simulink model "breakdown_FF"  (R2022b)
settings: Solver=VariableStepAuto  StartTime=0.0  StopTime=10.0  RelTol=1e-3
PreLoadFcn:
  | TOP;
undefined symbols (not defined in the file): ff_p, ff_z, p, r
libraries: dsparch4 x9, dspsrcs4 x4, dspspect3 x3, simulink_extras x3, dspmathops x3, cstblocks x2
settings Model: SimulationMode=accelerator  Creator=kschutz  LastModifiedBy=kschutz

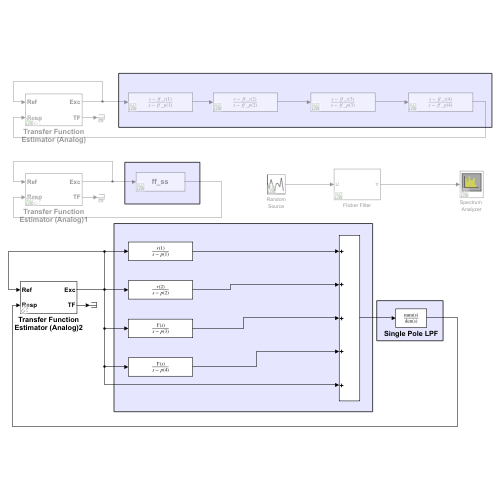
[thumbnail: Simulink's stored preview of the top-level diagram]
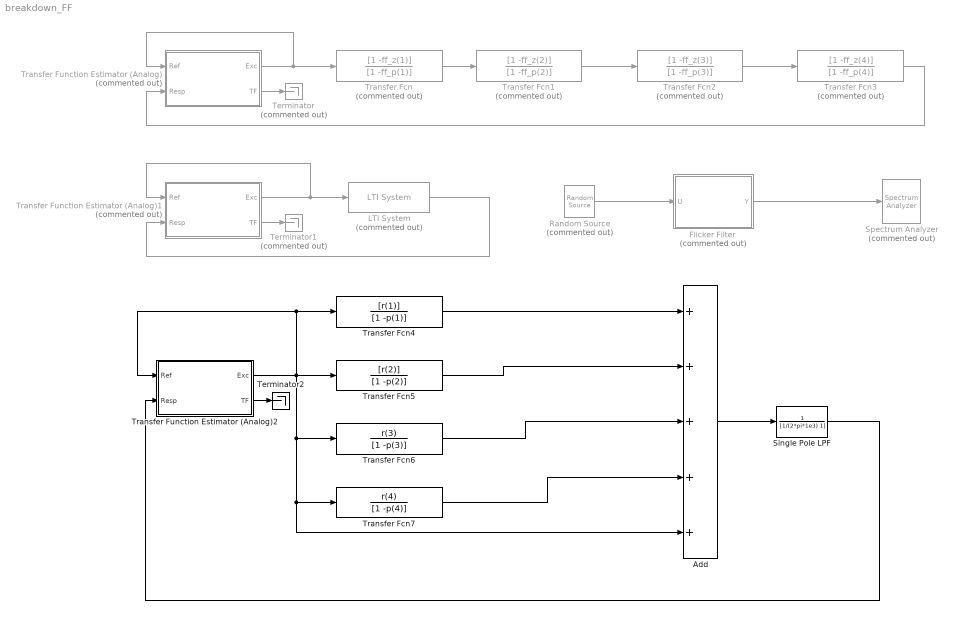
== system breakdown_FF ==
  Add : Sum  Inputs=+++++
  Flicker Filter : Subsystem  Commented=on
  LTI System : cstblocks/LTI System  Commented=on  sys=ff_ss  IC=[]
  Random Source : dspsrcs4/Random Source  Commented=on  SrcType=Uniform  NormMethod=Ziggurat  CltLength=12  MinVal=0  MaxVal=1  MeanVal=0  VarVal=1  RepMode=Not repeatable  rawSeed=1  IsInherit=off  SampMode=Discrete  SampTime=1e-5  SampFrame=1  DataType=Double  OutComplex=Real  OutputFrames=off
  Single Pole LPF : TransferFcn  Denominator=[1/(2*pi*1e3) 1]
  Spectrum Analyzer : SpectrumAnalyzer  Commented=on
  Terminator : Terminator  Commented=on
  Terminator1 : Terminator  Commented=on
  Terminator2 : Terminator
  Transfer Fcn : TransferFcn  Commented=on  Numerator=[1 -ff_z(1)]  Denominator=[1 -ff_p(1)]
  Transfer Fcn1 : TransferFcn  Commented=on  Numerator=[1 -ff_z(2)]  Denominator=[1 -ff_p(2)]
  Transfer Fcn2 : TransferFcn  Commented=on  Numerator=[1 -ff_z(3)]  Denominator=[1 -ff_p(3)]
  Transfer Fcn3 : TransferFcn  Commented=on  Numerator=[1 -ff_z(4)]  Denominator=[1 -ff_p(4)]
  Transfer Fcn4 : TransferFcn  Numerator=[r(1)]  Denominator=[1 -p(1)]
  Transfer Fcn5 : TransferFcn  Numerator=[r(2)]  Denominator=[1 -p(2)]
  Transfer Fcn6 : TransferFcn  Numerator=r(3)  Denominator=[1 -p(3)]
  Transfer Fcn7 : TransferFcn  Numerator=r(4)  Denominator=[1 -p(4)]
  Transfer Function Estimator (Analog) : Subsystem  Commented=on  AncestorBlock=|  mask(Baseband Analog Transfer Function Estimator){BW=100e3, Nfft=100e3, Navg=1, HoldOff=0}
      | Kblocks/Transfer Function
      | Estimator (Analog)
      mask prompts: BW "Bandwidth"; Nfft "FFT size"; Navg "Number of Averages"; HoldOff "Hold Off (seconds)"
      mask init:
      | % Select subset of FFT bins that are not aliased
      | % for output and display purposes.
      | % Said subset is based on the oversampling factor.
      | % Here we use a 2.56x oversampling factor.
      | % For example, for a 1024 point FFT size, the relatively
      | % alias free FFT bins would be bins 1 to 401.
      | % floor(1024/2.56) + 1 = 401.
      | OSR = 2.56;
      | AliasFree = floor(Nfft/OSR) + 1;
      settings: LibrarySourceBlock=|
      | Kblocks/Transfer Function
      | Estimator (Analog)
  Transfer Function Estimator (Analog)1 : Subsystem  Commented=on  AncestorBlock=|  mask(Baseband Analog Transfer Function Estimator){BW=100e3, Nfft=100e3, Navg=1, HoldOff=0}
      | Kblocks/Transfer Function
      | Estimator (Analog)
      mask prompts: BW "Bandwidth"; Nfft "FFT size"; Navg "Number of Averages"; HoldOff "Hold Off (seconds)"
      mask init: same as breakdown_FF/Transfer Function Estimator (Analog)
      settings: LibrarySourceBlock=|
      | Kblocks/Transfer Function
      | Estimator (Analog)
  Transfer Function Estimator (Analog)2 : Subsystem  AncestorBlock=|  mask(Baseband Analog Transfer Function Estimator){BW=100e3, Nfft=100e3, Navg=1, HoldOff=0}
      | Kblocks/Transfer Function
      | Estimator (Analog)
      mask prompts: BW "Bandwidth"; Nfft "FFT size"; Navg "Number of Averages"; HoldOff "Hold Off (seconds)"
      mask init: same as breakdown_FF/Transfer Function Estimator (Analog)
      settings: LibrarySourceBlock=|
      | Kblocks/Transfer Function
      | Estimator (Analog)
  wires:
  Transfer Fcn/1 -> Transfer Fcn1/1
  Transfer Fcn1/1 -> Transfer Fcn2/1
  Transfer Fcn2/1 -> Transfer Fcn3/1
  Transfer Function Estimator (Analog)/1(Exc) -> Transfer Function Estimator (Analog)/1(Ref), Transfer Fcn/1
  Transfer Fcn3/1 -> Transfer Function Estimator (Analog)/2(Resp)
  Transfer Function Estimator (Analog)1/1(Exc) -> Transfer Function Estimator (Analog)1/1(Ref), LTI System/1
  LTI System/1 -> Transfer Function Estimator (Analog)1/2(Resp)
  Transfer Function Estimator (Analog)2/1(Exc) -> Transfer Fcn7/1, Add/5, Transfer Fcn6/1, Transfer Fcn5/1, Transfer Fcn4/1, Transfer Function Estimator (Analog)2/1(Ref)
  Transfer Fcn4/1 -> Add/1
  Transfer Fcn5/1 -> Add/2
  Transfer Fcn6/1 -> Add/3
  Transfer Fcn7/1 -> Add/4
  Add/1 -> Single Pole LPF/1
  Single Pole LPF/1 -> Transfer Function Estimator (Analog)2/2(Resp)
  Transfer Function Estimator (Analog)/2(TF) -> Terminator/1
  Transfer Function Estimator (Analog)1/2(TF) -> Terminator1/1
  Transfer Function Estimator (Analog)2/2(TF) -> Terminator2/1
  Random Source/1 -> Flicker Filter/1(U)
  Flicker Filter/1(Y) -> Spectrum Analyzer/1

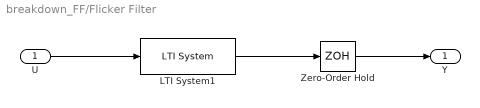
== system breakdown_FF/Flicker Filter ==
  U : Inport
  LTI System1 : cstblocks/LTI System  sys=ff_ss  IC=[]
  Zero-Order Hold : ZeroOrderHold  SampleTime=1e-5
  Y : Outport
  wires:
  Zero-Order Hold/1 -> Y/1
  LTI System1/1 -> Zero-Order Hold/1
  U/1 -> LTI System1/1

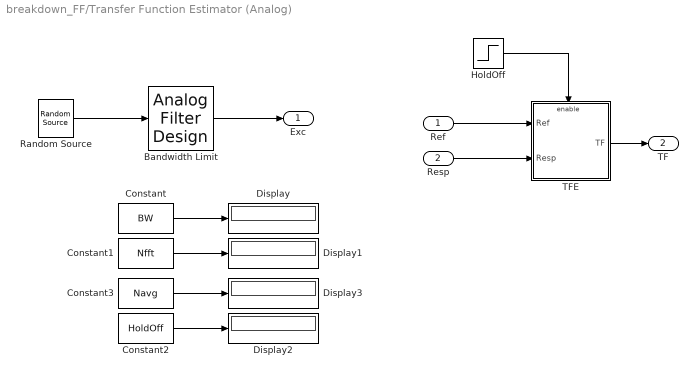
== system breakdown_FF/Transfer Function Estimator (Analog) ==
  Ref : Inport
  Resp : Inport  Port=2
  Bandwidth Limit : dsparch4/Analog Filter Design  method=Elliptic  filttype=Lowpass  N=8  Wlo=2*pi*BW  Whi=80  Rp=2  Rs=120
  Constant : Constant  Value=BW
  Constant1 : Constant  Value=Nfft
  Constant2 : Constant  Value=HoldOff
  Constant3 : Constant  Value=Navg
  Display{,1..3} (4 alike) : Display
  HoldOff : Step  Time=HoldOff  SampleTime=0
  Random Source : dspsrcs4/Random Source  SrcType=Uniform  NormMethod=Ziggurat  CltLength=12  MinVal=0  MaxVal=1  MeanVal=0  VarVal=1  RepMode=Specify seed  rawSeed=1  IsInherit=off  SampMode=Discrete  SampTime=1/(2.56*BW)  SampFrame=1  DataType=Double  OutComplex=Real  OutputFrames=off
  TFE : Subsystem
  Exc : Outport
  TF : Outport  Port=2
  wires:
  TFE/1(TF) -> TF/1
  Bandwidth Limit/1 -> Exc/1
  Random Source/1 -> Bandwidth Limit/1
  Constant1/1 -> Display1/1
  Constant2/1 -> Display2/1
  Constant/1 -> Display/1
  Ref/1 -> TFE/1(Ref)
  Resp/1 -> TFE/2(Resp)
  HoldOff/1 -> TFE/Enable
  Constant3/1 -> Display3/1

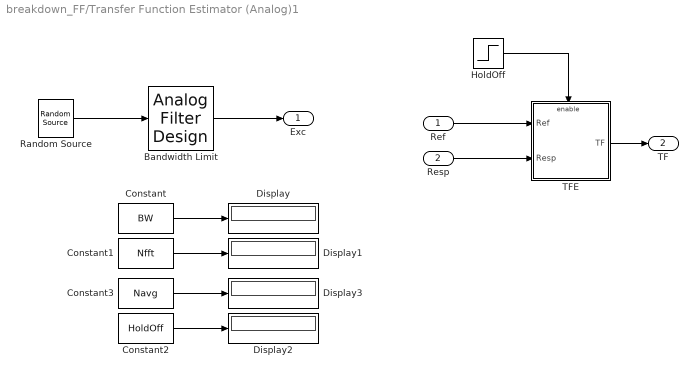
== system breakdown_FF/Transfer Function Estimator (Analog)1 ==
  Ref : Inport
  Resp : Inport  Port=2
  Bandwidth Limit : dsparch4/Analog Filter Design  method=Elliptic  filttype=Lowpass  N=8  Wlo=2*pi*BW  Whi=80  Rp=2  Rs=120
  Constant : Constant  Value=BW
  Constant1 : Constant  Value=Nfft
  Constant2 : Constant  Value=HoldOff
  Constant3 : Constant  Value=Navg
  Display{,1..3} (4 alike) : Display
  HoldOff : Step  Time=HoldOff  SampleTime=0
  Random Source : dspsrcs4/Random Source  SrcType=Uniform  NormMethod=Ziggurat  CltLength=12  MinVal=0  MaxVal=1  MeanVal=0  VarVal=1  RepMode=Specify seed  rawSeed=1  IsInherit=off  SampMode=Discrete  SampTime=1/(2.56*BW)  SampFrame=1  DataType=Double  OutComplex=Real  OutputFrames=off
  TFE : Subsystem
  Exc : Outport
  TF : Outport  Port=2
  wires:
  Constant3/1 -> Display3/1
  HoldOff/1 -> TFE/Enable
  Resp/1 -> TFE/2(Resp)
  Ref/1 -> TFE/1(Ref)
  Constant/1 -> Display/1
  Constant2/1 -> Display2/1
  Constant1/1 -> Display1/1
  Random Source/1 -> Bandwidth Limit/1
  Bandwidth Limit/1 -> Exc/1
  TFE/1(TF) -> TF/1

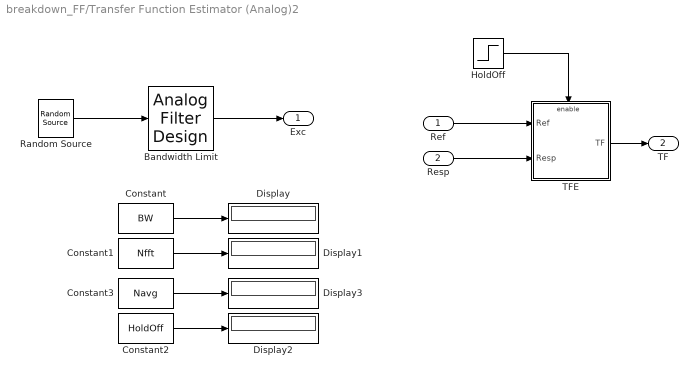
== system breakdown_FF/Transfer Function Estimator (Analog)2 ==
  Ref : Inport
  Resp : Inport  Port=2
  Bandwidth Limit : dsparch4/Analog Filter Design  method=Elliptic  filttype=Lowpass  N=8  Wlo=2*pi*BW  Whi=80  Rp=2  Rs=120
  Constant : Constant  Value=BW
  Constant1 : Constant  Value=Nfft
  Constant2 : Constant  Value=HoldOff
  Constant3 : Constant  Value=Navg
  Display{,1..3} (4 alike) : Display
  HoldOff : Step  Time=HoldOff  SampleTime=0
  Random Source : dspsrcs4/Random Source  SrcType=Uniform  NormMethod=Ziggurat  CltLength=12  MinVal=0  MaxVal=1  MeanVal=0  VarVal=1  RepMode=Specify seed  rawSeed=1  IsInherit=off  SampMode=Discrete  SampTime=1/(2.56*BW)  SampFrame=1  DataType=Double  OutComplex=Real  OutputFrames=off
  TFE : Subsystem
  Exc : Outport
  TF : Outport  Port=2
  wires:
  TFE/1(TF) -> TF/1
  Bandwidth Limit/1 -> Exc/1
  Random Source/1 -> Bandwidth Limit/1
  Constant1/1 -> Display1/1
  Constant2/1 -> Display2/1
  Constant/1 -> Display/1
  Ref/1 -> TFE/1(Ref)
  Resp/1 -> TFE/2(Resp)
  HoldOff/1 -> TFE/Enable
  Constant3/1 -> Display3/1

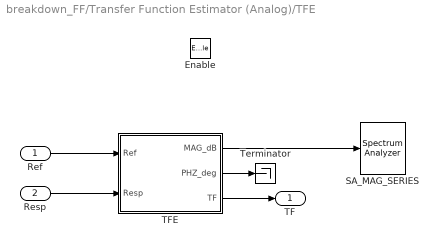
== system breakdown_FF/Transfer Function Estimator (Analog)/TFE ==
  Ref : Inport
  Resp : Inport  Port=2
  Enable : EnablePort
  SA_MAG_SERIES : SpectrumAnalyzer  IsFrequencyInputMode=1
  TFE : Subsystem
  Terminator : Terminator
  TF : Outport
  wires:
  TFE/3(TF) -> TF/1
  Resp/1 -> TFE/2(Resp)
  Ref/1 -> TFE/1(Ref)
  TFE/1(MAG_dB) -> SA_MAG_SERIES/1
  TFE/2(PHZ_deg) -> Terminator/1

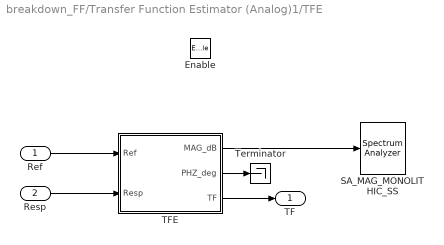
== system breakdown_FF/Transfer Function Estimator (Analog)1/TFE ==
  Ref : Inport
  Resp : Inport  Port=2
  Enable : EnablePort
  SA_MAG_MONOLITHIC_SS : SpectrumAnalyzer  IsFrequencyInputMode=1
  TFE : Subsystem
  Terminator : Terminator
  TF : Outport
  wires:
  TFE/1(MAG_dB) -> SA_MAG_MONOLITHIC_SS/1
  Ref/1 -> TFE/1(Ref)
  Resp/1 -> TFE/2(Resp)
  TFE/3(TF) -> TF/1
  TFE/2(PHZ_deg) -> Terminator/1

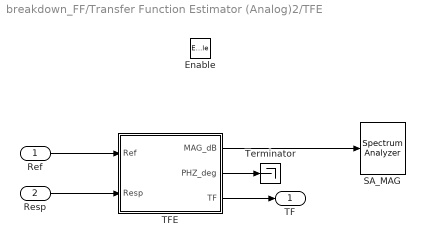
== system breakdown_FF/Transfer Function Estimator (Analog)2/TFE ==
  Ref : Inport
  Resp : Inport  Port=2
  Enable : EnablePort
  SA_MAG : SpectrumAnalyzer  IsFrequencyInputMode=1
  TFE : Subsystem
  Terminator : Terminator
  TF : Outport
  wires:
  TFE/3(TF) -> TF/1
  Resp/1 -> TFE/2(Resp)
  Ref/1 -> TFE/1(Ref)
  TFE/1(MAG_dB) -> SA_MAG/1
  TFE/2(PHZ_deg) -> Terminator/1

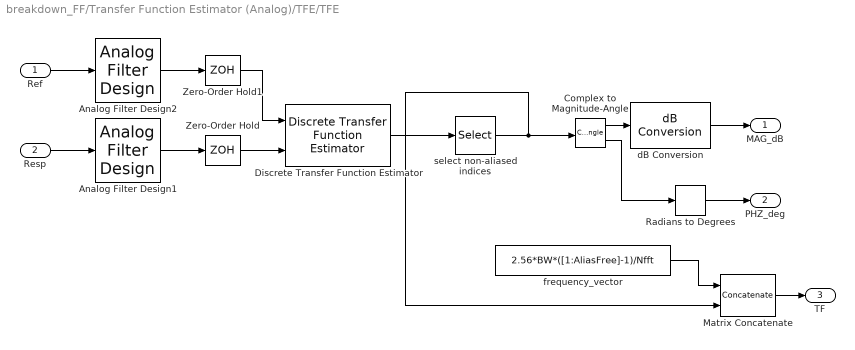
== system breakdown_FF/Transfer Function Estimator (Analog)/TFE/TFE ==
  Ref : Inport
  Resp : Inport  Port=2
  Analog Filter Design1 : dsparch4/Analog Filter Design  method=Elliptic  filttype=Lowpass  N=8  Wlo=2*pi*BW  Whi=80  Rp=2  Rs=100
  Analog Filter Design2 : dsparch4/Analog Filter Design  method=Elliptic  filttype=Lowpass  N=8  Wlo=2*pi*BW  Whi=80  Rp=2  Rs=100
  Complex to Magnitude-Angle : ComplexToMagnitudeAngle
  Discrete Transfer Function Estimator : dspspect3/Discrete Transfer Function Estimator  WindowMode=Specify on dialog  WindowLength=Nfft  Overlap=0  AveragingMethod=Running  ForgettingFactorPort=off  ForgettingFactor=0.9  SpectralAverages=Navg  FFTLengthSource=Property  FFTLength=Nfft  Window=Hann  SidelobeAttenuation=60  FrequencyRange=One-sided  OutputCoherence=off  SimulateUsing=Interpreted execution
  Matrix Concatenate : Concatenate  Mode=Multidimensional array  ConcatenateDimension=2
  Radians to Degrees : simulink_extras/Transformations/Radians to Degrees
  Zero-Order Hold : ZeroOrderHold  SampleTime=1/(OSR*BW)
  Zero-Order Hold1 : ZeroOrderHold  SampleTime=1/(OSR*BW)
  dB Conversion : dspmathops/dB Conversion  dBtype=dB  intype=Amplitude  R=1  fuzz=off
  frequency_vector : Constant  Value=2.56*BW*([1:AliasFree]-1)/Nfft
  select non-aliased indices : Selector  NumberOfDimensions=2  InputPortWidth=3  IndexOptions=Index vector (dialog),Select all  Indices=[1:AliasFree ],1  OutputSizes=1,1
  MAG_dB : Outport
  PHZ_deg : Outport  Port=2
  TF : Outport  Port=3
  wires:
  Matrix Concatenate/1 -> TF/1
  select non-aliased indices/1 -> Complex to Magnitude-Angle/1, Matrix Concatenate/2
  frequency_vector/1 -> Matrix Concatenate/1
  Discrete Transfer Function Estimator/1 -> select non-aliased indices/1
  Complex to Magnitude-Angle/2 -> Radians to Degrees/1
  Analog Filter Design1/1 -> Zero-Order Hold/1
  Analog Filter Design2/1 -> Zero-Order Hold1/1
  Radians to Degrees/1 -> PHZ_deg/1
  dB Conversion/1 -> MAG_dB/1
  Resp/1 -> Analog Filter Design1/1
  Zero-Order Hold1/1 -> Discrete Transfer Function Estimator/1
  Ref/1 -> Analog Filter Design2/1
  Complex to Magnitude-Angle/1 -> dB Conversion/1
  Zero-Order Hold/1 -> Discrete Transfer Function Estimator/2

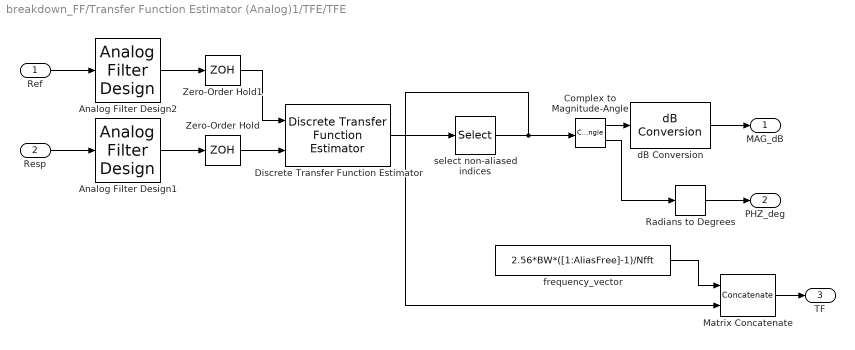
== system breakdown_FF/Transfer Function Estimator (Analog)1/TFE/TFE ==
  Ref : Inport
  Resp : Inport  Port=2
  Analog Filter Design1 : dsparch4/Analog Filter Design  method=Elliptic  filttype=Lowpass  N=8  Wlo=2*pi*BW  Whi=80  Rp=2  Rs=100
  Analog Filter Design2 : dsparch4/Analog Filter Design  method=Elliptic  filttype=Lowpass  N=8  Wlo=2*pi*BW  Whi=80  Rp=2  Rs=100
  Complex to Magnitude-Angle : ComplexToMagnitudeAngle
  Discrete Transfer Function Estimator : dspspect3/Discrete Transfer Function Estimator  WindowMode=Specify on dialog  WindowLength=Nfft  Overlap=0  AveragingMethod=Running  ForgettingFactorPort=off  ForgettingFactor=0.9  SpectralAverages=Navg  FFTLengthSource=Property  FFTLength=Nfft  Window=Hann  SidelobeAttenuation=60  FrequencyRange=One-sided  OutputCoherence=off  SimulateUsing=Interpreted execution
  Matrix Concatenate : Concatenate  Mode=Multidimensional array  ConcatenateDimension=2
  Radians to Degrees : simulink_extras/Transformations/Radians to Degrees
  Zero-Order Hold : ZeroOrderHold  SampleTime=1/(OSR*BW)
  Zero-Order Hold1 : ZeroOrderHold  SampleTime=1/(OSR*BW)
  dB Conversion : dspmathops/dB Conversion  dBtype=dB  intype=Amplitude  R=1  fuzz=off
  frequency_vector : Constant  Value=2.56*BW*([1:AliasFree]-1)/Nfft
  select non-aliased indices : Selector  NumberOfDimensions=2  InputPortWidth=3  IndexOptions=Index vector (dialog),Select all  Indices=[1:AliasFree ],1  OutputSizes=1,1
  MAG_dB : Outport
  PHZ_deg : Outport  Port=2
  TF : Outport  Port=3
  wires:
  Zero-Order Hold/1 -> Discrete Transfer Function Estimator/2
  Complex to Magnitude-Angle/1 -> dB Conversion/1
  Ref/1 -> Analog Filter Design2/1
  Zero-Order Hold1/1 -> Discrete Transfer Function Estimator/1
  Resp/1 -> Analog Filter Design1/1
  dB Conversion/1 -> MAG_dB/1
  Radians to Degrees/1 -> PHZ_deg/1
  Analog Filter Design2/1 -> Zero-Order Hold1/1
  Analog Filter Design1/1 -> Zero-Order Hold/1
  Complex to Magnitude-Angle/2 -> Radians to Degrees/1
  Discrete Transfer Function Estimator/1 -> select non-aliased indices/1
  frequency_vector/1 -> Matrix Concatenate/1
  select non-aliased indices/1 -> Matrix Concatenate/2, Complex to Magnitude-Angle/1
  Matrix Concatenate/1 -> TF/1

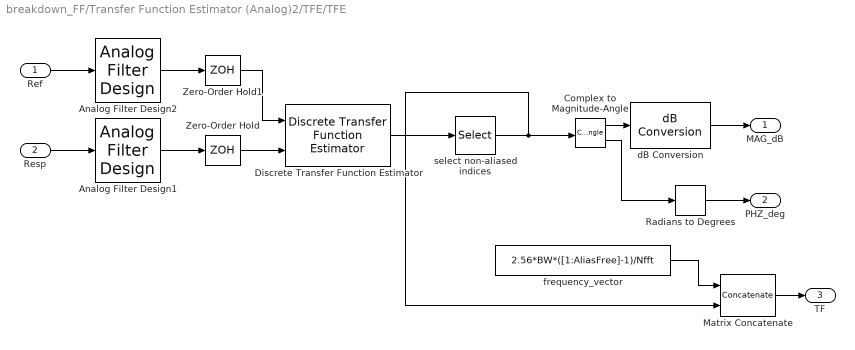
== system breakdown_FF/Transfer Function Estimator (Analog)2/TFE/TFE ==
  Ref : Inport
  Resp : Inport  Port=2
  Analog Filter Design1 : dsparch4/Analog Filter Design  method=Elliptic  filttype=Lowpass  N=8  Wlo=2*pi*BW  Whi=80  Rp=2  Rs=100
  Analog Filter Design2 : dsparch4/Analog Filter Design  method=Elliptic  filttype=Lowpass  N=8  Wlo=2*pi*BW  Whi=80  Rp=2  Rs=100
  Complex to Magnitude-Angle : ComplexToMagnitudeAngle
  Discrete Transfer Function Estimator : dspspect3/Discrete Transfer Function Estimator  WindowMode=Specify on dialog  WindowLength=Nfft  Overlap=0  AveragingMethod=Running  ForgettingFactorPort=off  ForgettingFactor=0.9  SpectralAverages=Navg  FFTLengthSource=Property  FFTLength=Nfft  Window=Hann  SidelobeAttenuation=60  FrequencyRange=One-sided  OutputCoherence=off  SimulateUsing=Interpreted execution
  Matrix Concatenate : Concatenate  Mode=Multidimensional array  ConcatenateDimension=2
  Radians to Degrees : simulink_extras/Transformations/Radians to Degrees
  Zero-Order Hold : ZeroOrderHold  SampleTime=1/(OSR*BW)
  Zero-Order Hold1 : ZeroOrderHold  SampleTime=1/(OSR*BW)
  dB Conversion : dspmathops/dB Conversion  dBtype=dB  intype=Amplitude  R=1  fuzz=off
  frequency_vector : Constant  Value=2.56*BW*([1:AliasFree]-1)/Nfft
  select non-aliased indices : Selector  NumberOfDimensions=2  InputPortWidth=3  IndexOptions=Index vector (dialog),Select all  Indices=[1:AliasFree ],1  OutputSizes=1,1
  MAG_dB : Outport
  PHZ_deg : Outport  Port=2
  TF : Outport  Port=3
  wires:
  Matrix Concatenate/1 -> TF/1
  select non-aliased indices/1 -> Complex to Magnitude-Angle/1, Matrix Concatenate/2
  frequency_vector/1 -> Matrix Concatenate/1
  Discrete Transfer Function Estimator/1 -> select non-aliased indices/1
  Complex to Magnitude-Angle/2 -> Radians to Degrees/1
  Analog Filter Design1/1 -> Zero-Order Hold/1
  Analog Filter Design2/1 -> Zero-Order Hold1/1
  Radians to Degrees/1 -> PHZ_deg/1
  dB Conversion/1 -> MAG_dB/1
  Resp/1 -> Analog Filter Design1/1
  Zero-Order Hold1/1 -> Discrete Transfer Function Estimator/1
  Ref/1 -> Analog Filter Design2/1
  Complex to Magnitude-Angle/1 -> dB Conversion/1
  Zero-Order Hold/1 -> Discrete Transfer Function Estimator/2
